simulink model "complete_model"  (R2024b)
settings: Solver=ode5  StartTime=0.0  StopTime=2.509  MaxStep=1/512000  RelTol=1e-3  AbsTol=1e-6
values from neighbouring files (symbols this model uses):
  fM = fM_vector(j)    [tradeoff.m]
  r = 2 * round(r_target / 2)    [tradeoff.m]
undefined symbols (not defined in the file or in its folder): DiscIntNeverNeededParam
libraries: simulink_extras x2
settings Model: SimulationMode=rapid-accelerator  ExtModeTrigDuration=100  Creator=The MathWorks, Inc.  LastModifiedBy=himes
settings SolverCC: AutoScaleAbsTol=off  AlgebraicLoopSolver=TrustRegion  MaxZcPerStep=1
settings DataIOCC: SaveFinalState=on  SaveFormat=Array  SaveOutput=off  SaveState=on  ReturnWorkspaceOutputs=off  StateSaveName=tmp_raccel_xout  TimeSaveName=tmp_raccel_tout  SignalLoggingName=tmp_raccel_logsout
settings OptimizationCC: BlockReduction=off  BooleanDataType=off  ExpressionDepthLimit=2147483647  RollThreshold=2  InitFltsAndDblsToZero=on  EfficientMapNaN2IntZero=off  LifeSpan=inf  SimCompilerOptimization=on
settings DebuggingCC: SaveWithParameterizedLinksMsg=none  UnderspecifiedInitializationDetection=Classic  MergeDetectMultiDrivingBlocksExec=none  SignalResolutionControl=TryResolveAllWithWarning  MultiTaskDSMMsg=warning  MultiTaskCondExecSysMsg=none  IntegerOverflowMsg=none  FcnCallInpInsideContextMsg=warning  UnconnectedInputMsg=warning  UnconnectedOutputMsg=warning  UnconnectedLineMsg=warning  AllowSymbolicDim=off  StateNameClashWarn=warning  SymbolicDimsDataTypeCodeGenerationDiagnostic=none  SFUnexpectedBacktrackingDiag=warning  SFNoUnconditionalDefaultTransitionDiag=warning  SFExecutionAtInitializationDiag=none  IntegerSaturationMsg=none  ArithmeticOperatorsInVariantConditions=warning
settings HardwareCC: ProdBitPerPointer=32  ProdBitPerSizeT=32  ProdBitPerPtrDiffT=32  ProdLargestAtomicFloat=None  ProdIntDivRoundTo=Undefined  ProdEndianess=Unspecified  ProdWordSize=32  ProdHWDeviceType=32-bit Generic  TargetBitPerPointer=64  TargetBitPerSizeT=64  TargetBitPerPtrDiffT=64  TargetLongLongMode=on  TargetIntDivRoundTo=Zero  TargetEndianess=LittleEndian  TargetWordSize=64  TargetHWDeviceType=MATLAB Host  ProdEqTarget=off
settings ModelReferenceCC: EnableRefExpFcnMdlSchedulingChecks=on  PropagateSignalLabelsOutOfModel=off
settings SFSimCC: SimUseLocalCustomCode=off  CustomCodeUndefinedFunction=UseInterfaceOnly
settings RTWCC: SystemTargetFile=raccel.tlc  TemplateMakefile=raccel_default_tmf  RTWVerbose=off  RTWUseLocalCustomCode=off  RTWUseSimCustomCode=on  CustomBLASCallback=coder.internal.blas.MATLABBLASCallback
settings CodeAppCC: GenerateComments=off  MaxIdLength=128  MangleLength=10  SimulinkBlockComments=off
settings RaccelTargetCC: TargetLangStandard=C99 (ISO)  InstructionSetFMA=off  OptimizeReductions=off  LogToMDFFile=off  ENABLE_SLEXEC_SSBRIDGE=1  RTWCAPIParams=on  RTWCAPIRootIO=on
settings ConfigComp: CovMetricSettings=dw  CovSaveCumulativeToWorkspaceVar=on  CovSaveSingleToWorkspaceVar=on  CovExternalEMLEnable=off

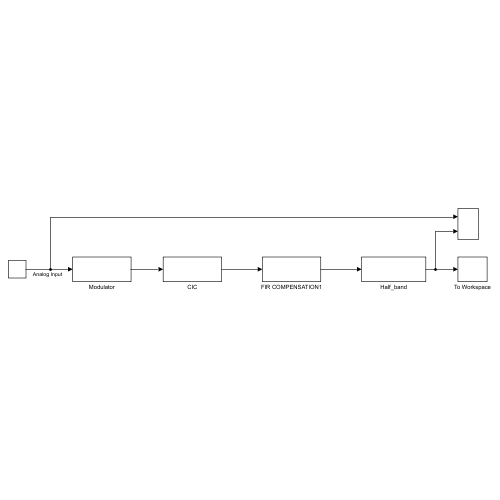
[thumbnail: Simulink's stored preview of the top-level diagram]
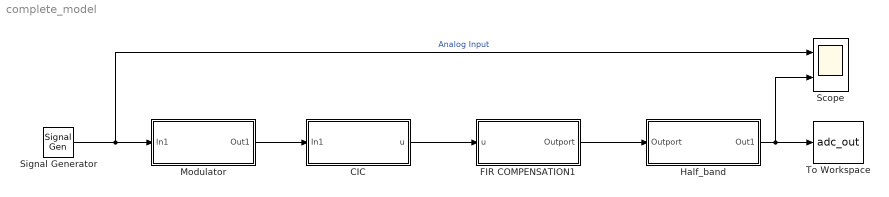
== system complete_model ==
  CIC : Subsystem
  FIR COMPENSATION1 : Subsystem
  Half_band : Subsystem
  Modulator : Subsystem
  Scope : Scope  NumInputPorts=2
  Signal Generator : SignalGenerator  Frequency=100
  To Workspace : ToWorkspace  VariableName=adc_out  SampleTime=-1
      settings: Save2DSignal=2-D array (concatenate along first dimension)
  wires:
  Signal Generator/1 -> Modulator/1(In1), Scope/1  "Analog Input"
  Modulator/1(Out1) -> CIC/1(In1)
  FIR COMPENSATION1/1(Outport) -> Half_band/1(Outport)
  Half_band/1(Out1) -> Scope/2, To Workspace/1
  CIC/1(u) -> FIR COMPENSATION1/1(u)

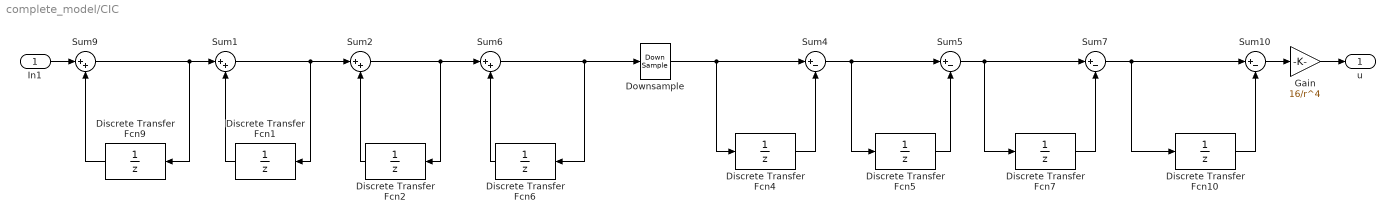
== system complete_model/CIC ==
  In1 : Inport
  Discrete Transfer Fcn{1..2,4..7,9..10} (8 alike) : DiscreteTransferFcn  Denominator=[1 0]
  Downsample : DownSample  N=r  RateOptions=Allow multirate processing
  Gain : Gain  Gain=16/r^4
  Sum{1..2,6,9} (4 alike) : Sum  Inputs=|++
  Sum{4..5,7,10} (4 alike) : Sum  Inputs=|+-
  u : Outport
  wires:
  Sum7/1 -> Sum10/1, Discrete Transfer Fcn10/1
  Discrete Transfer Fcn10/1 -> Sum10/2
  Downsample/1 -> Discrete Transfer Fcn4/1, Sum4/1
  Discrete Transfer Fcn5/1 -> Sum5/2
  Sum1/1 -> Sum2/1, Discrete Transfer Fcn1/1
  Discrete Transfer Fcn1/1 -> Sum1/2
  Discrete Transfer Fcn2/1 -> Sum2/2
  Sum5/1 -> Sum7/1, Discrete Transfer Fcn7/1
  Sum4/1 -> Sum5/1, Discrete Transfer Fcn5/1
  Discrete Transfer Fcn9/1 -> Sum9/2
  In1/1 -> Sum9/1
  Sum9/1 -> Sum1/1, Discrete Transfer Fcn9/1
  Sum6/1 -> Downsample/1, Discrete Transfer Fcn6/1
  Discrete Transfer Fcn6/1 -> Sum6/2
  Gain/1 -> u/1
  Sum2/1 -> Sum6/1, Discrete Transfer Fcn2/1
  Discrete Transfer Fcn4/1 -> Sum4/2
  Discrete Transfer Fcn7/1 -> Sum7/2
  Sum10/1 -> Gain/1

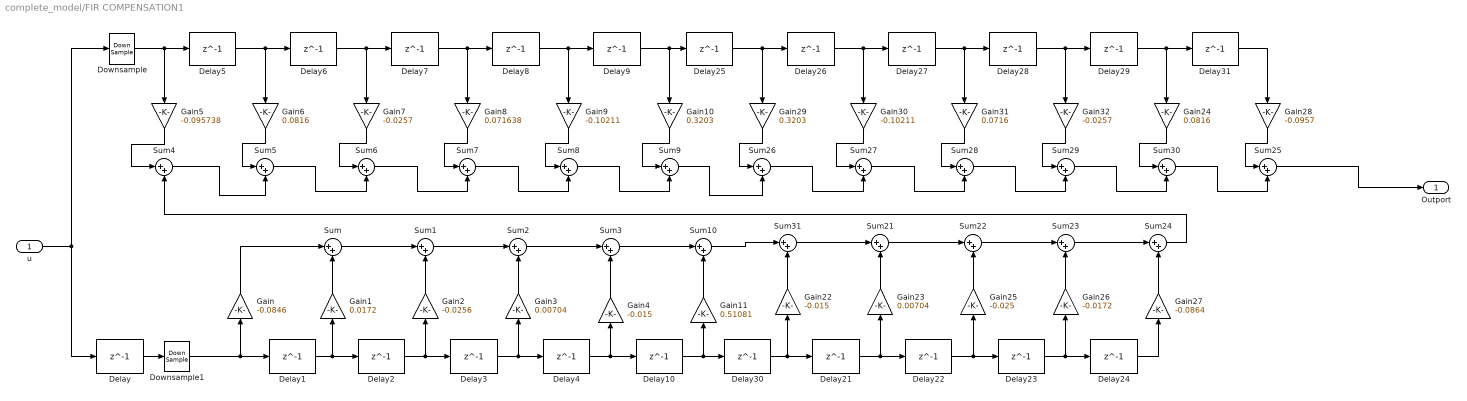
== system complete_model/FIR COMPENSATION1 ==
  u : Inport
  Delay{,1..10,21..31} (22 alike) : Delay  DelayLength=1  InitialCondition=0  UseCircularBuffer=on
  Downsample : DownSample  N=1  RateOptions=Allow multirate processing
  Downsample1 : DownSample  N=1  RateOptions=Allow multirate processing
  Gain : Gain  Gain=-0.0846
  Gain1 : Gain  Gain=0.0172
  Gain10 : Gain  Gain=0.3203
  Gain11 : Gain  Gain=0.51081
  Gain2 : Gain  Gain=-0.0256
  Gain22 : Gain  Gain=-0.015
  Gain23 : Gain  Gain=0.00704
  Gain24 : Gain  Gain=0.0816
  Gain25 : Gain  Gain=-0.025
  Gain26 : Gain  Gain=-0.0172
  Gain27 : Gain  Gain=-0.0864
  Gain28 : Gain  Gain=-0.0957
  Gain29 : Gain  Gain=0.3203
  Gain3 : Gain  Gain=0.00704
  Gain30 : Gain  Gain=-0.10211
  Gain31 : Gain  Gain=0.0716
  Gain32 : Gain  Gain=-0.0257
  Gain4 : Gain  Gain=-0.015
  Gain5 : Gain  Gain=-0.095738
  Gain6 : Gain  Gain=0.0816
  Gain7 : Gain  Gain=-0.0257
  Gain8 : Gain  Gain=0.071638
  Gain9 : Gain  Gain=-0.10211
  Sum{,1..10,21..31} (22 alike) : Sum  Inputs=|++
  Outport : Outport
  wires:
  Sum7/1 -> Sum8/2
  Delay2/1 -> Gain2/1, Delay3/1
  Gain29/1 -> Sum26/1
  Delay28/1 -> Gain32/1, Delay29/1
  Gain25/1 -> Sum22/2
  Sum23/1 -> Sum24/1
  Delay1/1 -> Gain1/1, Delay2/1
  Delay3/1 -> Gain3/1, Delay4/1
  Gain10/1 -> Sum9/1
  Sum31/1 -> Sum21/1
  Sum30/1 -> Sum25/2
  Delay31/1 -> Gain28/1
  Sum8/1 -> Sum9/2
  Delay4/1 -> Gain4/1, Delay10/1
  Gain7/1 -> Sum6/1
  Delay5/1 -> Gain6/1, Delay6/1
  Delay/1 -> Downsample1/1
  Sum6/1 -> Sum7/2
  Delay6/1 -> Gain7/1, Delay7/1
  Delay8/1 -> Gain9/1, Delay9/1
  Gain5/1 -> Sum4/1
  Gain8/1 -> Sum7/1
  Gain4/1 -> Sum3/2
  Sum1/1 -> Sum2/1
  Gain1/1 -> Sum/2
  Sum5/1 -> Sum6/2
  Gain6/1 -> Sum5/1
  Sum2/1 -> Sum3/1
  Delay29/1 -> Gain24/1, Delay31/1
  Sum3/1 -> Sum10/1
  Gain28/1 -> Sum25/1
  Sum21/1 -> Sum22/1
  Delay23/1 -> Gain26/1, Delay24/1
  Sum25/1 -> Outport/1
  Delay22/1 -> Gain25/1, Delay23/1
  Sum10/1 -> Sum31/1
  Sum9/1 -> Sum26/2
  Delay30/1 -> Gain22/1, Delay21/1
  Gain/1 -> Sum/1
  Gain22/1 -> Sum31/2
  Gain27/1 -> Sum24/2
  Gain11/1 -> Sum10/2
  Gain23/1 -> Sum21/2
  Delay24/1 -> Gain27/1
  Sum26/1 -> Sum27/2
  Delay10/1 -> Gain11/1, Delay30/1
  Gain24/1 -> Sum30/1
  Gain30/1 -> Sum27/1
  Sum/1 -> Sum1/1
  Sum29/1 -> Sum30/2
  Sum4/1 -> Sum5/2
  Delay21/1 -> Gain23/1, Delay22/1
  Sum24/1 -> Sum4/2
  Gain3/1 -> Sum2/2
  Gain2/1 -> Sum1/2
  Gain26/1 -> Sum23/2
  Gain9/1 -> Sum8/1
  Sum27/1 -> Sum28/2
  Gain32/1 -> Sum29/1
  Delay26/1 -> Gain30/1, Delay27/1
  Delay25/1 -> Gain29/1, Delay26/1
  Downsample1/1 -> Delay1/1, Gain/1
  Delay7/1 -> Gain8/1, Delay8/1
  Sum22/1 -> Sum23/1
  Gain31/1 -> Sum28/1
  Delay9/1 -> Delay25/1, Gain10/1
  u/1 -> Downsample/1, Delay/1
  Sum28/1 -> Sum29/2
  Delay27/1 -> Gain31/1, Delay28/1
  Downsample/1 -> Gain5/1, Delay5/1

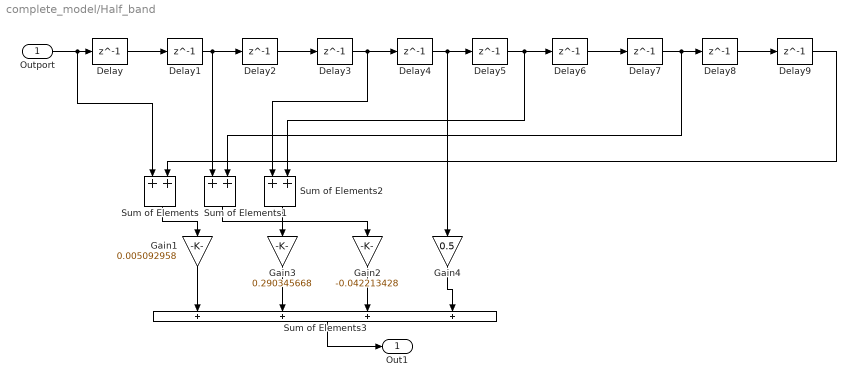
== system complete_model/Half_band ==
  Outport : Inport
  Delay{,1..9} (10 alike) : Delay  DelayLength=1  InitialCondition=0  UseCircularBuffer=on
  Gain1 : Gain  Gain=0.005092958
  Gain2 : Gain  Gain=-0.042213428
  Gain3 : Gain  Gain=0.290345668
  Gain4 : Gain  Gain=0.5
  Sum of Elements : Sum
  Sum of Elements1 : Sum
  Sum of Elements2 : Sum
  Sum of Elements3 : Sum  Inputs=++++
  Out1 : Outport
  wires:
  Delay9/1 -> Sum of Elements/2
  Sum of Elements3/1 -> Out1/1
  Delay3/1 -> Sum of Elements2/1, Delay4/1
  Delay4/1 -> Gain4/1, Delay5/1
  Delay5/1 -> Sum of Elements2/2, Delay6/1
  Delay6/1 -> Delay7/1
  Delay1/1 -> Delay2/1, Sum of Elements1/1
  Sum of Elements/1 -> Gain1/1
  Gain2/1 -> Sum of Elements3/3
  Gain1/1 -> Sum of Elements3/1
  Sum of Elements1/1 -> Gain2/1
  Gain3/1 -> Sum of Elements3/2
  Sum of Elements2/1 -> Gain3/1
  Delay/1 -> Delay1/1
  Delay7/1 -> Sum of Elements1/2, Delay8/1
  Gain4/1 -> Sum of Elements3/4
  Delay8/1 -> Delay9/1
  Delay2/1 -> Delay3/1
  Outport/1 -> Sum of Elements/1, Delay/1

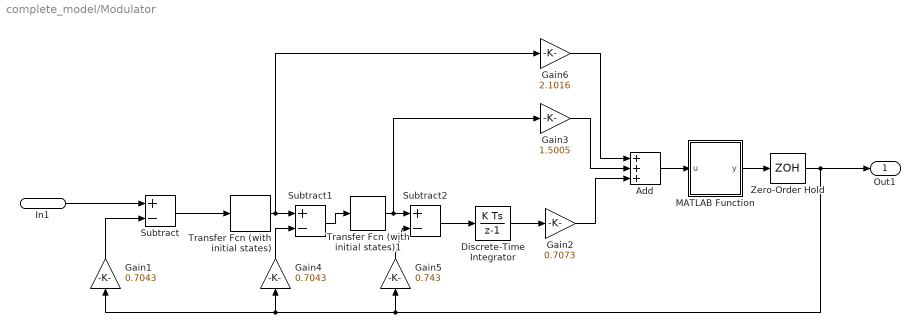
== system complete_model/Modulator ==
  In1 : Inport
  Add : Sum  Inputs=+++
  Discrete-Time Integrator : DiscreteIntegrator  gainval=1  SampleTime=1/fM  UpperSaturationLimit=+2  LowerSaturationLimit=-2  ICPrevOutput=DiscIntNeverNeededParam  ICPrevScaledInput=DiscIntNeverNeededParam
  Gain1 : Gain  Gain=0.7043
  Gain2 : Gain  Gain=0.7073
  Gain3 : Gain  Gain=1.5005
  Gain4 : Gain  Gain=0.7043
  Gain5 : Gain  Gain=0.743
  Gain6 : Gain  Gain=2.1016
  MATLAB Function : MATLAB Function  TreatAsAtomicUnit=on
  Subtract : Sum  Inputs=+-
  Subtract1 : Sum  Inputs=+-
  Subtract2 : Sum  Inputs=+-
  Transfer Fcn (with initial states) : simulink_extras/Additional Linear/Transfer Fcn (with initial states)  N=[1]  D=[1 0]  X0=0
  Transfer Fcn (with initial states)1 : simulink_extras/Additional Linear/Transfer Fcn (with initial states)  N=[1]  D=[1 0]  X0=0
  Zero-Order Hold : ZeroOrderHold  SampleTime=1/fM
  Out1 : Outport
  wires:
  Subtract/1 -> Transfer Fcn (with initial states)/1
  Gain1/1 -> Subtract/2
  Gain2/1 -> Add/3
  Gain3/1 -> Add/2
  In1/1 -> Subtract/1
  Gain6/1 -> Add/1
  Zero-Order Hold/1 -> Out1/1, Gain5/1, Gain4/1, Gain1/1
  Transfer Fcn (with initial states)/1 -> Subtract1/1, Gain6/1
  MATLAB Function/1(y) -> Zero-Order Hold/1
  Add/1 -> MATLAB Function/1(u)
  Subtract1/1 -> Transfer Fcn (with initial states)1/1
  Discrete-Time Integrator/1 -> Gain2/1
  Transfer Fcn (with initial states)1/1 -> Gain3/1, Subtract2/1
  Subtract2/1 -> Discrete-Time Integrator/1
  Gain4/1 -> Subtract1/2
  Gain5/1 -> Subtract2/2

== matlab function complete_model/Modulator/MATLAB Function ==
  data: u input; y output
function y = fcn(u)
    if u >= 0
        y = 1.8;
    else 
        y = -1.8;
    end
